simulink model "motor_diagrama_sim"  (R2026a)
settings: Solver=VariableStepAuto  StopTime=1
settings Model: Creator=juand  LastModifiedBy=juand

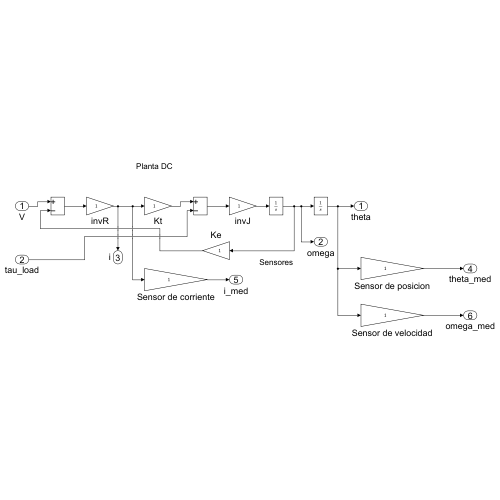
[thumbnail: Simulink's stored preview of the top-level diagram]
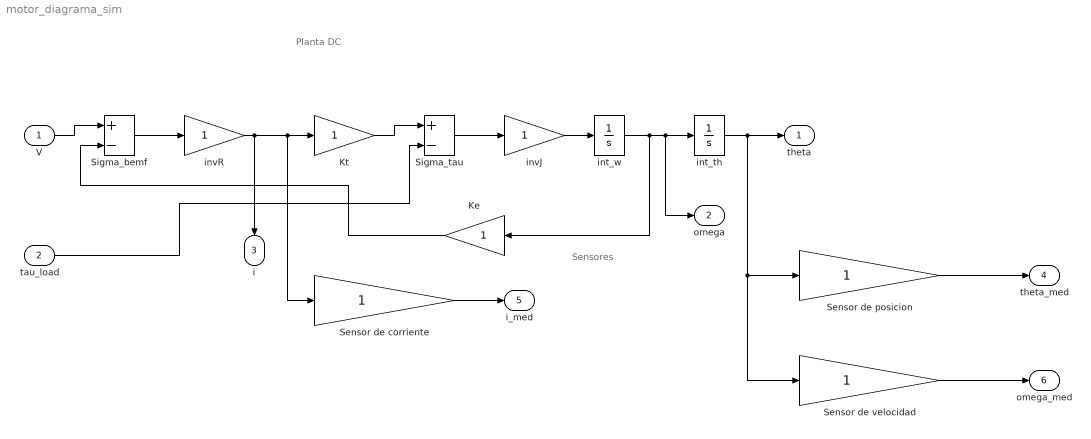
== system motor_diagrama_sim ==
  note: Planta DC
  note: Sensores
  V : Inport
  tau_load : Inport  Port=2
  Ke : Gain
  Kt : Gain
  Sensor de corriente : Gain
  Sensor de posicion : Gain
  Sensor de velocidad : Gain
  Sigma_bemf : Sum  Inputs=+-
  Sigma_tau : Sum  Inputs=+-
  int_th : Integrator
  int_w : Integrator
  invJ : Gain
  invR : Gain
  theta : Outport
  omega : Outport  Port=2
  i : Outport  Port=3
  theta_med : Outport  Port=4
  i_med : Outport  Port=5
  omega_med : Outport  Port=6
  wires:
  V/1 -> Sigma_bemf/1
  Sigma_bemf/1 -> invR/1
  invR/1 -> Kt/1, Sensor de corriente/1, i/1
  Kt/1 -> Sigma_tau/1
  tau_load/1 -> Sigma_tau/2
  Sigma_tau/1 -> invJ/1
  invJ/1 -> int_w/1
  int_w/1 -> int_th/1, omega/1, Ke/1
  Ke/1 -> Sigma_bemf/2
  int_th/1 -> Sensor de velocidad/1, Sensor de posicion/1, theta/1
  Sensor de posicion/1 -> theta_med/1
  Sensor de corriente/1 -> i_med/1
  Sensor de velocidad/1 -> omega_med/1
